simulink model "testrig_quarter_car_doublewishbone"  (R2025a)
settings: Solver=ode23t  StartTime=0.0  StopTime=309  MaxStep=0.01  RelTol=1e-3  AbsTol=1e-3  EnableMultiTasking=on
PostLoadFcn:
  | Vehicle_data_dwishbone;Maneuver = sm_car_maneuverdata_knc(0.19,-0.21,0.01,1.3,0.1,500,1200,1200,1200,1200,-0.3);
values from neighbouring files (symbols this model uses):
  Vehicle = evalin('base','Vehicle')    [sm_car_knc_plot1toecamber.m]
undefined symbols (not defined in the file or in its folder): X, Y, Z
libraries: sm_lib x9, sm_car_testrig_utilities_lib x5, nesl_utility x4, fl_lib x2, Damper_Linear x1, Linkage_DW_B x1, Spring_Linear x1, Suspension_Utilities x1
CloseFcn:
  | clear simlog_sm_car_testrig_quarter_car
  | clear logsout_sm_car_testrig_quarter_car
Description:
  | Quarter Car Testrig, Pushrod Upper Arm
  | 
  | Copyright 2021-2026 The MathWorks, Inc.
settings Model: Creator=smiller  LastModifiedBy=smiller
settings SolverCC: AutoScaleAbsTol=off  AlgebraicLoopSolver=TrustRegion
settings DataIOCC: LimitDataPoints=on  MaxDataPoints=10000  ReturnWorkspaceOutputs=off  SignalLoggingName=logsout_sm_car_testrig_quarter_car
settings OptimizationCC: ReuseModelBlockBuffer=off  LifeSpan=inf
settings DebuggingCC: UnconnectedInputMsg=warning  UnconnectedOutputMsg=warning  UnconnectedLineMsg=warning  AllowSymbolicDim=off  SFUnexpectedBacktrackingDiag=warning  SFNoUnconditionalDefaultTransitionDiag=warning  SFExecutionAtInitializationDiag=none  ArithmeticOperatorsInVariantConditions=warning
settings ModelReferenceCC: EnableRefExpFcnMdlSchedulingChecks=on
settings SFSimCC: SimUseLocalCustomCode=off  CustomCodeUndefinedFunction=UseInterfaceOnly
settings RTWCC: RTWUseLocalCustomCode=off  GPUComputeCapability=3.5
settings CodeAppCC: StateflowObjectComments=on
settings GRTTargetCC: TargetLangStandard=C89/C90 (ANSI)
settings ConfigComp: CovMetricSettings=dw  CovSaveCumulativeToWorkspaceVar=on  CovSaveSingleToWorkspaceVar=on  CovExternalEMLEnable=off  CovSFcnEnable=off
settings SimscapeCC: SimscapeLogType=all  SimscapeLogSimulationStatistics=on  SimscapeLogName=simlog_sm_car_testrig_quarter_car  SimscapeLogLimitData=off  SimscapeLogDataHistory=10000.0
settings DiagnosticsConfigSet: SimMechanicsUnconnectedFramePorts=none
settings ExplorerConfigSet: InternalSimMechanicsExplorerSettings="<ExplorerConfiguration><canonicalview>default</canonicalview><AnimationSetting><BasePlaybackSpeed>1.0</BasePlaybackSpeed><PlaybackSpeedFactor>16.0</PlaybackSpeedFactor></AnimationSetting><TilePanel><TileInfo><Tiles Columns=\"1\" Count=\"1\" Rows=\"1\"><Column Weight=\"1\"/><Row Weight=\"1\"/><Tile Height=\"1\" Width=\"1\" X=\"0\" Y=\"0\"/></Tiles></TileInfo><SceneInfo><SceneViewer><BGColor><R>1</R><G>1</G><B>1</B></BGColor><Camera><DoPerspective>off</DoPerspective><Position><X>0.609546959525912757</X><Y>-0.12768849868824983</Y><Z>0.743207391319535282</Z></Position><Center><X>0.032196690336286915</X><Y>0.449661770501376012</Y><Z>0.16585712212990944</Z></Center><Up><X>-0.408248290463863073</X><Y>0.408248290463863073</Y><Z>0.816496580927726145</Z></Up><ViewLimDist>1</ViewLimDist><YLim>0.584271163693107387</YLim><XLim>0.685764276635102643</XLim></Camera></SceneViewer></SceneInfo></TilePanel><MechEditorPanel><Cameras/><GfxPanelCameraMap/><VideoCreator><PlaybackSpeedRatio>1.0</PlaybackSpeedRatio><FrameRate>30</FrameRate><VideoFormat>Motion JPEG AVI</VideoFormat><FrameSize>auto</FrameSize></VideoCreator></MechEditorPanel></ExplorerConfiguration>"

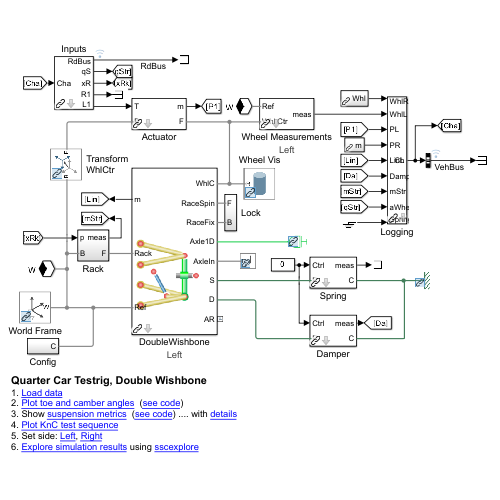
[thumbnail: Simulink's stored preview of the top-level diagram]
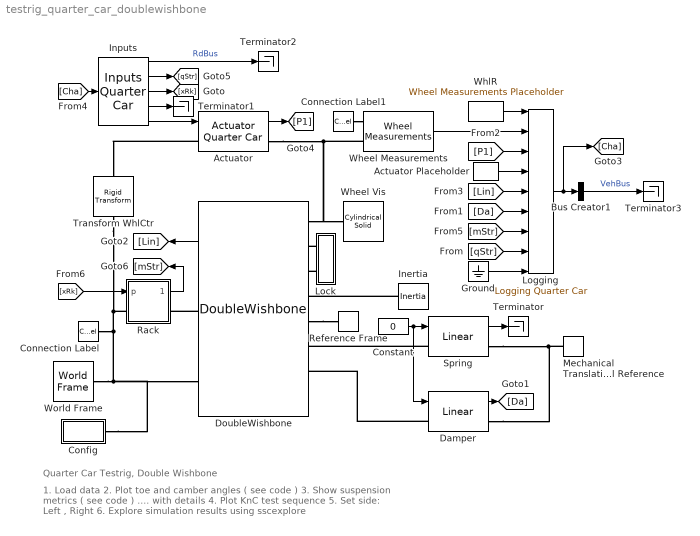
== system testrig_quarter_car_doublewishbone ==
  note: Quarter Car Testrig, Double Wishbone
  note: 1. Load data
      | 2. Plot toe and camber angles ( see code )
      | 3. Show suspension metrics ( see code ) .... with details
      | 4. Plot KnC test sequence
      | 5. Set side: Left , Right
      | 6. Explore simulation results using sscexplore
  Actuator : sm_car_testrig_utilities_lib/Actuator Quarter Car  veh=Vehicle  xCPOffset=Maneuver.xCPOffset
  Actuator Placeholder : sm_car_testrig_utilities_lib/Actuator Placeholder  SystemSampleTime=-1  VariantActivationTime=update diagram  EmptyChoice=off  PassThrough=off  PassThroughVariantControl=(default)  EmptyChoiceVariantControl=(default)  AllowFlexibleInterface=on  Latency=0  AutoFrameSizeCalculation=off
  Bus Creator1 : BusCreator  Inputs=1
  Config : Subsystem
  Connection Label : ConnectionLabel  Label=W
  Connection Label1 : ConnectionLabel  Label=W
  Constant : Constant  Value=0
  Damper : Damper_Linear/Linear  VariantControl=Linear  dam_b=Vehicle.Chassis.Damper.Axle1.Damping.d.Value  hp_dpr_top=Vehicle.Chassis.Damper.Axle1.Damping.sTop.Value  hp_dpr_bot=Vehicle.Chassis.Damper.Axle1.Damping.sBottom.Value  bs_lim_upper=Vehicle.Chassis.Damper.Axle1.Endstop.xMax.Value  bs_lim_lower=Vehicle.Chassis.Damper.Axle1.Endstop.xMin.Value  bs_k_upper=Vehicle.Chassis.Damper.Axle1.Endstop.KxMax.Value  bs_k_lower=Vehicle.Chassis.Damper.Axle1.Endstop.KxMin.Value  bs_b_upper=Vehicle.Chassis.Damper.Axle1.Endstop.dxMax.Value  bs_b_lower=Vehicle.Chassis.Damper.Axle1.Endstop.dxMin.Value  bs_region=Vehicle.Chassis.Damper.Axle1.Endstop.xTransition.Value
  DoubleWishbone : Linkage_DW_B/DoubleWishbone  VariantControl=DoubleWishbone  popup_leftRight=Left  hp_in_f_ua=Vehicle.Chassis.SuspA1.Linkage.UpperWishbone.sInboardF.Value  hp_in_r_ua=Vehicle.Chassis.SuspA1.Linkage.UpperWishbone.sInboardR.Value  hp_out_ua=Vehicle.Chassis.SuspA1.Linkage.UpperWishbone.sOutboard.Value  hp_in_f_la=Vehicle.Chassis.SuspA1.Linkage.LowerWishbone.sInboardF.Value  hp_in_r_la=Vehicle.Chassis.SuspA1.Linkage.LowerWishbone.sInboardR.Value  hp_out_la=Vehicle.Chassis.SuspA1.Linkage.LowerWishbone.sOutboard.Value  hp_arb=Vehicle.Chassis.SuspA1.Linkage.LowerWishbone.sARB.Value  hp_upr_cg=Vehicle.Chassis.SuspA1.Linkage.Upright.sCG.Value  hp_upr_wc=Vehicle.Chassis.SuspA1.Linkage.Upright.sWheelCentre.Value  hp_in_rod=Vehicle.Chassis.SuspA1.Linkage.TrackRod.sInboard.Value  hp_upr_rod=Vehicle.Chassis.SuspA1.Linkage.TrackRod.sOutboard.Value  hp_spr_top=Vehicle.Chassis.SuspA1.Linkage.Shock.sTop.Value  hp_spr_bot=Vehicle.Chassis.SuspA1.Linkage.Shock.sBottom.Value  clr_hp=Visual.hp.clr  opc_hp=Visual.hp.opc  size_hp=Visual.hp.rad  Upper_Arm_to_Subframe=Vehicle.Chassis.SuspA1.Linkage.Upper_Arm_to_Subframe  ua_mass=Vehicle.Chassis.SuspA1.Linkage.UpperWishbone.m.Value  clr_ua=Visual.UpperArm.clr  opc_ua=Visual.part.opc  radius_ua=Visual.UpperArm.rad  Lower_Arm_to_Subframe=Vehicle.Chassis.SuspA1.Linkage.Lower_Arm_to_Subframe  arm_mass=Vehicle.Chassis.SuspA1.Linkage.LowerWishbone.m.Value  clr_la=Visual.LowerArm.clr  opc_la=Visual.part.opc  radius_la=Visual.LowerArm.rad  shock_pist_mass=Vehicle.Chassis.SuspA1.Linkage.Shock.mPiston.Value  shock_cyl_mass=Vehicle.Chassis.SuspA1.Linkage.Shock.mCylinder.Value  up_lim_bumpstop=Vehicle.Chassis.SuspA1.Linkage.Endstop.xMax.Value  low_lim_bumpstop=Vehicle.Chassis.SuspA1.Linkage.Endstop.xMin.Value  clr_conn_shock=Visual.hp.clr  opc_conn_shock=Visual.hp.opc  size_conn_shock=Visual.hp.rad  clr_shock_cyl=Visual.Shock.cyl.clr  opc_shock_cyl=Visual.part.opc  radius_shock_cyl=Visual.Shock.cyl.rad  clr_shock_piston=Visual.Shock.piston.clr  opc_shock_piston=Visual.part.opc  clr_shock_bumpstop=Visual.Shock.bumpstop.clr  opc_shock_bumpstop=Visual.part.opc  deadvol_len_shock_cyl=Visual.Shock.dead_length  piston_len_shock=Visual.Shock.piston.len  cyl_cap_len_shock=Visual.Shock.cap.len  bumpstop_len_shock=Visual.Shock.bumpstop.len  upr_mass=Vehicle.Chassis.SuspA1.Linkage.Upright.m.Value  atoe=Vehicle.Chassis.SuspA1.Linkage.Upright.aToe.Value  acamber=Vehicle.Chassis.SuspA1.Linkage.Upright.aCamber.Value  axle_len=Vehicle.Chassis.SuspA1.Linkage.Upright.xAxle.Value  axle_whlc_to_bearing=Vehicle.Chassis.SuspA1.Linkage.Upright.xWCtoBearing.Value  axle_mass=Vehicle.Chassis.SuspA1.Linkage.Upright.mAxle.Value  clr_conn_upr=Visual.hp.clr  opc_conn_upr=Visual.hp.opc  size_conn_upr=Visual.hp.rad  clr_upr=Visual.Upright.clr  opc_upr=Visual.part.opc  radius_upr=Visual.Upright.rad  clr_axle=Visual.Axle.clr  opc_axle=Visual.part.opc  radius_axle=Visual.Axle.rad  rod_mass=Vehicle.Chassis.SuspA1.Linkage.TrackRod.m.Value  clr_conn_rod=Visual.hp.clr  opc_conn_rod=Visual.hp.opc  size_conn_rod=Visual.hp.rad  clr_rod=Visual.TrackRod.clr  opc_rod=Visual.part.opc  radius_rod=Visual.TrackRod.rad  whl_init_spd_lr=Init.Axle1.nWheel.Value
      settings: AttributesFormatString=%<popup_leftRight>
  Ground : Ground
  Inertia : fl_lib/Mechanical/Rotational Elements/Inertia  inertia=0.01 kg*m^2  num_ports=foundation.enum.numPorts2.one  w_specify=on  w_priority=None  w=0 rad/s  w_nominal_specify=off  w_nominal_value=1  w_nominal_unit=rad/s  t_specify=off  t_priority=None  t=0 N*m  t_nominal_specify=off  t_nominal_value=1  t_nominal_unit=N*m
  Inputs : sm_car_testrig_utilities_lib/Inputs Quarter Car  popup_steering_input=On
  Lock : Subsystem
  Logging : sm_car_testrig_utilities_lib/Logging Quarter Car
  Mechanical Translational Reference : fl_lib/Mechanical/Translational Elements/Mechanical Translational Reference
  Rack : Subsystem
  Reference Frame : sm_lib/Frames and Transforms/Reference Frame
  Spring : Spring_Linear/Linear  VariantControl=Linear  spr_def0=Vehicle.Chassis.Spring.Axle1.xPreload.Value  spr_frc0=Vehicle.Chassis.Spring.Axle1.fPreload.Value  spr_k=Vehicle.Chassis.Spring.Axle1.K.Value  spr_hp_top=Vehicle.Chassis.Spring.Axle1.sTop.Value  spr_hp_bot=Vehicle.Chassis.Spring.Axle1.sBottom.Value
  Terminator{,1..3} (4 alike) : Terminator
  Transform WhlCtr : sm_lib/Frames and Transforms/Rigid Transform  RotationMethod=None  FollAlignAxisA=+X  BaseAlignAxisA=+Y  FollAlignAxisB=+Y  BaseAlignAxisB=+Z  RotationStandardAxis=+Z  RotationAngle=0.0  RotationAngleUnits=deg  RotationArbitraryAxis=[0 0 1]  RotationSequenceAxes=FollowerAxes  RotationSequence=XYX  RotationSequenceAngles=[0 0 0]  RotationSequenceAnglesUnits=deg  RotationMatrix=[1 0 0; 0 1 0; 0 0 1]  Quaternion=[1 0 0 0]  TranslationMethod=StandardAxis  TranslationCartesianOffset=[0 0 0]  TranslationCartesianOffsetUnits=m  TranslationStandardAxis=+Z  TranslationStandardOffset=Vehicle.Chassis.SuspA1.Linkage.Upright.sWheelCentre.Value(3)  TranslationStandardOffsetUnits=m  TranslationROffset=0  TranslationROffsetUnits=m  TranslationThetaOffset=0  TranslationThetaOffsetUnits=deg  TranslationZOffset=0  TranslationZOffsetUnits=m
  Wheel Measurements : Suspension_Utilities/Wheel Measurements  popup_leftRight=Left
      settings: AttributesFormatString=%<popup_leftRight>
  Wheel Vis : sm_lib/Body Elements/Cylindrical Solid  CylinderRadius=0.23  CylinderRadiusUnits=m  CylinderLength=0.25  CylinderLengthUnits=m  ExportEntireGeometry=off  InertiaType=CalculateFromGeometry  BasedOnType=Mass  Density=1000  DensityUnits=kg/m^3  Mass=10  MassUnits=kg  CenterOfMass=[0 0 0]  CenterOfMassUnits=m  MomentsOfInertia=[1 1 1]  MomentsOfInertiaUnits=kg*m^2  ProductsOfInertia=[0 0 0]  ProductsOfInertiaUnits=kg*m^2  GraphicType=FromGeometry  MarkerShape=Sphere  MarkerSize=10  GraphicVisPropType=SimpleVisualProperties  GraphicDiffuseColor=[0.5 0.5 0.5]  GraphicOpacity=0.3  GraphicSpecularColor=[0.5 0.5 0.5 1.0]  GraphicAmbientColor=[0.15 0.15 0.15 1.0]  GraphicEmissiveColor=[0.0 0.0 0.0 1.0]  GraphicShininess=75  DoExposeReferenceFrame=on  SerializedFrames=<Frames/>
  WhlR : sm_car_testrig_utilities_lib/Wheel Measurements Placeholder  SystemSampleTime=-1  VariantActivationTime=update diagram  EmptyChoice=off  PassThrough=off  PassThroughVariantControl=(default)  EmptyChoiceVariantControl=(default)  AllowFlexibleInterface=on  Latency=0  AutoFrameSizeCalculation=off
  World Frame : sm_lib/Frames and Transforms/World Frame
  wires:
  Damper/1 -> [Da]
  Constant/1 -> Damper/1, Spring/1
  Spring/1 -> Terminator/1
  DoubleWishbone/1 -> [Lin]
  Actuator/1 -> [P1]
  [xRk] -> Rack/1(p)
  Inputs/1 -> Terminator2/1  "RdBus"
  Inputs/3 -> [xRk]
  Inputs/4 -> Terminator1/1
  [Cha] -> Inputs/1
  Inputs/2 -> [qStr]
  Inputs/5 -> Actuator/1
  Actuator Placeholder/1 -> Logging/4
  [qStr] -> Logging/8
  [Da] -> Logging/6
  [P1] -> Logging/3
  WhlR/1 -> Logging/1
  [Lin] -> Logging/5
  [mStr] -> Logging/7
  Ground/1 -> Logging/9
  Bus Creator1/1 -> Terminator3/1  "VehBus"
  Logging/1 -> [Cha], Bus Creator1/1
  Wheel Measurements/1 -> Logging/2
  Rack/1(meas) -> [mStr]
  connections:
  Wheel Vis/RConn1 -- DoubleWishbone/LConn1 -- Actuator/RConn1 -- Wheel Measurements/LConn2
  Mechanical Translational Reference/LConn1 -- Spring/RConn1 -- Damper/RConn1
  Actuator/LConn1 -- Transform WhlCtr/RConn1
  Spring/LConn1 -- DoubleWishbone/LConn6
  Inertia/LConn1 -- DoubleWishbone/LConn4
  DoubleWishbone/LConn5 -- Reference Frame/RConn1
  Damper/LConn1 -- DoubleWishbone/LConn7
  DoubleWishbone/RConn1 -- Rack/RConn1
  Connection Label/LConn1 -- World Frame/RConn1 -- Config/RConn1 -- DoubleWishbone/RConn2 -- Rack/LConn1 -- Transform WhlCtr/LConn1
  Connection Label1/LConn1 -- Wheel Measurements/LConn1
  Lock/LConn1 -- DoubleWishbone/LConn2
  Lock/LConn2 -- DoubleWishbone/LConn3

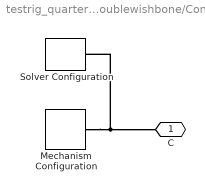
== system testrig_quarter_car_doublewishbone/Config ==
  Mechanism Configuration : sm_lib/Utilities/Mechanism Configuration  UniformGravity=Constant  GravityVector=[0 0 -9.80665]  GravityVectorUnits=m/s^2  LinearizationDelta=0.001  JointModeTransitionNonlinearIterations=2
  Solver Configuration : nesl_utility/Solver Configuration  PhysicalDomain=network_engine_domain  SubClassName=solver  LeftPortType=input  RightPortType=generic  Tones=[]  Harmonics=[]  SimulateNoise=off  Profile=off  UseLocalSampling=off  EnableSwitchedLinearOptims=on  FrequencyDomain=off  UseCCode=off  RelTol=0.001  AbsTol=1e-06  MinStep=1e-09  ToWorkspace=off  RevertToSquareIcSolve=off  NumHomotopyIterations=100  PhasorMode=off  PhasorModeNumHarmonics=1  ConsistencySolver=NEWTON_FTOL  IndexReductionMethod=DerivativeReplacement  DoDC=off  ResidualTolerance=1e-09  ConsistencyTolSource=GLOBAL  ConsistencyAbsTol=0.001  ConsistencyRelTol=0.001  ConsistencyTolFactor=0.001  UseLocalSolver=off  LocalSolverChoice=NE_BACKWARD_EULER_ADVANCER  ResolveIndetEquations=on  FunctionEvalNumThread=1  LocalSolverSampleTime=0.001  DoFixedCost=off  MaxNonlinIter=3  MaxModeIter=2  ComputeImpulses=off  ImpulseIterations=2  LinearAlgebra=Sparse  LinearAlgebraNumThread=0  EquationFormulation=NE_TIME_EF  DelaysMemoryBudget=1024  AutomaticFiltering=on  FilteringTimeConstant=0.001  PartitionStorageMethod=AS_NEEDED  PartitionMemoryBudget=1024  PartitionMethod=FAST  MultibodyUseLocalSolver=off  MultibodyLocalSolverChoice=ODE1  MultibodyLocalSolverSampleTime=0.001
  C : PMIOPort  Side=Right
  connections:
  Mechanism Configuration/RConn1 -- Solver Configuration/RConn1 -- C/RConn1

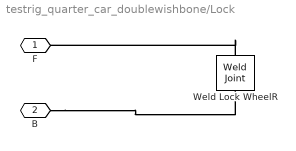
== system testrig_quarter_car_doublewishbone/Lock ==
  Weld Lock WheelR : sm_lib/Joints/Weld Joint  JointMode=Normal  CompositeWrenchDir=FollowerOnBase  CompositeWrenchFrame=BaseFrame  SenseConstraintForce=off  SenseConstraintTorque=off  SenseTotalForce=off  SenseTotalTorque=off
  F : PMIOPort  Side=Left
  B : PMIOPort  Port=2  Side=Left
  connections:
  B/RConn1 -- Weld Lock WheelR/LConn1
  Weld Lock WheelR/RConn1 -- F/RConn1

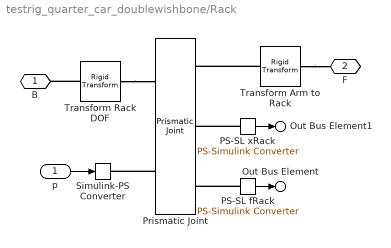
== system testrig_quarter_car_doublewishbone/Rack ==
  p : Inport
  PS-SL fRack : nesl_utility/PS-Simulink Converter  PhysicalDomain=network_engine_domain  SubClassName=ps_output  LeftPortType=input  RightPortType=output  PseudoPeriodic=off  Frequencies=[]  VectorFormat=1-D array  Unit=1  AffineConversion=off
  PS-SL xRack : nesl_utility/PS-Simulink Converter  PhysicalDomain=network_engine_domain  SubClassName=ps_output  LeftPortType=input  RightPortType=output  PseudoPeriodic=off  Frequencies=[]  VectorFormat=1-D array  Unit=1  AffineConversion=off
  Prismatic Joint : sm_lib/Joints/Prismatic Joint  JointMode=Normal  CompositeWrenchDir=FollowerOnBase  CompositeWrenchFrame=BaseFrame  SenseConstraintForce=off  SenseConstraintTorque=off  SenseTotalForce=off  SenseTotalTorque=off  PositionTargetSpecify=on  PositionTargetPriority=High  PositionTargetValue=0  PositionTargetValueUnits=m  VelocityTargetSpecify=off  VelocityTargetPriority=High  VelocityTargetValue=0  VelocityTargetValueUnits=m/s  EquilibriumPosition=0  EquilibriumPositionUnits=m  SpringStiffness=0  SpringStiffnessUnits=N/m  DampingCoefficient=0  DampingCoefficientUnits=N/(m/s)  LowerLimitSpecify=off  LowerLimitBound=-1  LowerLimitBoundUnits=m  LowerLimitStiffness=1e6  LowerLimitStiffnessUnits=N/m  LowerLimitDamping=1e3  LowerLimitDampingUnits=N/(m/s)  LowerLimitTransitionRegionWidth=1e-4  LowerLimitTransitionRegionWidthUnits=m  UpperLimitSpecify=off  UpperLimitBound=1  UpperLimitBoundUnits=m  UpperLimitStiffness=1e6  UpperLimitStiffnessUnits=N/m  UpperLimitDamping=1e3  UpperLimitDampingUnits=N/(m/s)  UpperLimitTransitionRegionWidth=1e-4  UpperLimitTransitionRegionWidthUnits=m  TorqueActuationMode=ComputedTorque  MotionActuationMode=InputMotion  SensePosition=on  SenseVelocity=off  SenseAcceleration=off  SenseTorqueForce=on  SenseLowerLimitTorqueForce=off  SenseUpperLimitTorqueForce=off
  Simulink-PS Converter : nesl_utility/Simulink-PS Converter  PhysicalDomain=network_engine_domain  SubClassName=ps_input  LeftPortType=input  RightPortType=output  PseudoPeriodic=off  Frequencies=[]  NoiseDistribution=none  NoiseParameters=[]  Unit=m  AffineConversion=off  FilteringAndDerivatives=filter  SimscapeFilterOrder=2  InputFilterTimeConstant=0.005  UdotUserProvided=0
  Transform Arm to Rack : sm_lib/Frames and Transforms/Rigid Transform  RotationMethod=StandardAxis  FollAlignAxisA=+X  BaseAlignAxisA=+Y  FollAlignAxisB=+Y  BaseAlignAxisB=+Z  RotationStandardAxis=+X  RotationAngle=90  RotationAngleUnits=deg  RotationArbitraryAxis=[0 0 1]  RotationSequenceAxes=FollowerAxes  RotationSequence=XYX  RotationSequenceAngles=[0 0 0]  RotationSequenceAnglesUnits=deg  RotationMatrix=[1 0 0; 0 1 0; 0 0 1]  Quaternion=[1 0 0 0]  TranslationMethod=Cartesian  TranslationCartesianOffset=Vehicle.Chassis.SuspA1.Linkage.TrackRod.sInboard.Value.*[1 0 1]  TranslationCartesianOffsetUnits=m  TranslationStandardAxis=+Z  TranslationStandardOffset=0  TranslationStandardOffsetUnits=m  TranslationROffset=0  TranslationROffsetUnits=m  TranslationThetaOffset=0  TranslationThetaOffsetUnits=deg  TranslationZOffset=0  TranslationZOffsetUnits=m
  Transform Rack DOF : sm_lib/Frames and Transforms/Rigid Transform  RotationMethod=StandardAxis  FollAlignAxisA=+X  BaseAlignAxisA=+Y  FollAlignAxisB=+Y  BaseAlignAxisB=+Z  RotationStandardAxis=+X  RotationAngle=90  RotationAngleUnits=deg  RotationArbitraryAxis=[0 0 1]  RotationSequenceAxes=FollowerAxes  RotationSequence=XYX  RotationSequenceAngles=[0 0 0]  RotationSequenceAnglesUnits=deg  RotationMatrix=[1 0 0; 0 1 0; 0 0 1]  Quaternion=[1 0 0 0]  TranslationMethod=Cartesian  TranslationCartesianOffset=Vehicle.Chassis.SuspA1.Linkage.TrackRod.sInboard.Value.*[1 0 1]  TranslationCartesianOffsetUnits=m  TranslationStandardAxis=+Z  TranslationStandardOffset=0  TranslationStandardOffsetUnits=m  TranslationROffset=0  TranslationROffsetUnits=m  TranslationThetaOffset=0  TranslationThetaOffsetUnits=deg  TranslationZOffset=0  TranslationZOffsetUnits=m
  B : PMIOPort  Side=Left
  F : PMIOPort  Port=2  Side=Right
  Out Bus Element : Outport  VectorParamsAs1DForOutWhenUnconnected=off  PortName=meas  Element=FRack
  Out Bus Element1 : Outport  VectorParamsAs1DForOutWhenUnconnected=off  PortName=meas  Element=xRack
  wires:
  p/1 -> Simulink-PS Converter/1
  PS-SL fRack/1 -> Out Bus Element/1
  PS-SL xRack/1 -> Out Bus Element1/1
  connections:
  Transform Rack DOF/RConn1 -- Prismatic Joint/LConn1
  Prismatic Joint/LConn2 -- Simulink-PS Converter/RConn1
  Transform Arm to Rack/LConn1 -- F/RConn1
  Transform Arm to Rack/RConn1 -- Prismatic Joint/RConn1
  Transform Rack DOF/LConn1 -- B/RConn1
  PS-SL xRack/LConn1 -- Prismatic Joint/RConn2
  PS-SL fRack/LConn1 -- Prismatic Joint/RConn3
